simulink model "BMS_4S1P"  (R2026a)
settings: Solver=VariableStepAuto  StopTime=600
libraries: fl_lib x20, nesl_utility x15, simulink x3, BMS_4S1P_ExternalBalancing_lib_lib x1, BatteryBalancing x1, BatteryEstimators x1
settings Model: Creator=jack2  LastModifiedBy=jack2

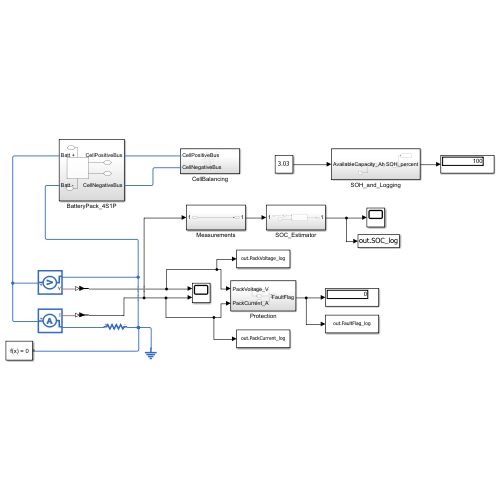
[thumbnail: Simulink's stored preview of the top-level diagram]
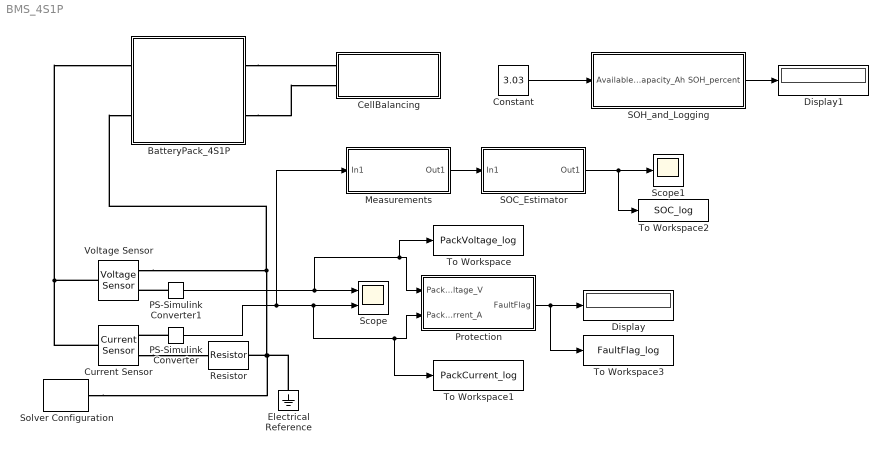
== system BMS_4S1P ==
  BatteryPack_4S1P : Subsystem
  CellBalancing : Subsystem
  Constant : Constant  Value=3.03
  Current Sensor : fl_lib/Electrical/Electrical Sensors/Current Sensor
  Display : Display
  Display1 : Display
  Electrical Reference : fl_lib/Electrical/Electrical Elements/Electrical Reference
  Measurements : Subsystem
  PS-Simulink Converter : nesl_utility/PS-Simulink Converter  PhysicalDomain=network_engine_domain  SubClassName=ps_output  LeftPortType=input  RightPortType=output  PseudoPeriodic=off  Frequencies=[]  VectorFormat=inherit  Unit=A  AffineConversion=off
  PS-Simulink Converter1 : nesl_utility/PS-Simulink Converter  PhysicalDomain=network_engine_domain  SubClassName=ps_output  LeftPortType=input  RightPortType=output  PseudoPeriodic=off  Frequencies=[]  VectorFormat=inherit  Unit=V  AffineConversion=off
  Protection : Subsystem
  Resistor : fl_lib/Electrical/Electrical Elements/Resistor  R=20 Ohm  i_specify=off  i_priority=None  i=0 A  i_nominal_specify=off  i_nominal_value=1  i_nominal_unit=A  v_specify=off  v_priority=None  v=0 V  v_nominal_specify=off  v_nominal_value=1  v_nominal_unit=V
  SOC_Estimator : Subsystem
  SOH_and_Logging : Subsystem
  Scope : Scope  NumInputPorts=2
      settings: ActiveDisplayYMinimum=2.7734819938047579  ActiveDisplayYMaximum=17.948779649470726
  Scope1 : Scope
      settings: ActiveDisplayYMinimum=0.77520540586084219  ActiveDisplayYMaximum=0.832743677575157
  Solver Configuration : nesl_utility/Solver Configuration  PhysicalDomain=network_engine_domain  SubClassName=solver  LeftPortType=input  RightPortType=generic  Tones=[]  Harmonics=[]  SimulateNoise=off  Profile=off  UseLocalSampling=off  EnableSwitchedLinearOptims=on  FrequencyDomain=off  UseCCode=off  RelTol=0.001  AbsTol=0.001  MinStep=1e-09  ToWorkspace=off  RevertToSquareIcSolve=off  NumHomotopyIterations=100  PhasorMode=off  PhasorModeNumHarmonics=1  ConsistencySolver=NEWTON_XTOL_AFTER_FTOL  CanonicalOrdering=CANONICAL  OptimizeIntermediates=OPTIMIZED  IndexReductionMethod=DerivativeReplacement  DoDC=off  ResidualTolerance=1e-09  ConsistencyTolSource=GLOBAL  ConsistencyAbsTol=0.001  ConsistencyRelTol=0.001  ConsistencyTolFactor=0.001  UseLocalSolver=off  LocalSolverChoice=NE_BACKWARD_EULER_ADVANCER  ResolveIndetEquations=on  FunctionEvalNumThread=1  LocalSolverSampleTime=0.001  DoFixedCost=off  MaxNonlinIter=3  MaxModeIter=2  ComputeImpulses=off  ImpulseIterations=2  LinearAlgebra=auto  LinearAlgebraNumThread=0  EquationFormulation=NE_TIME_EF  DelaysMemoryBudget=1024  AutomaticFiltering=on  FilteringTimeConstant=0.001  PartitionStorageMethod=AS_NEEDED  PartitionMemoryBudget=1024  PartitionMethod=ROBUST  MultibodyUseLocalSolver=off  MultibodyLocalSolverChoice=ODE1  MultibodyLocalSolverSampleTime=0.001
  To Workspace : ToWorkspace  VariableName=PackVoltage_log  SaveFormat=Timeseries  SampleTime=-1
  To Workspace1 : ToWorkspace  VariableName=PackCurrent_log  SaveFormat=Timeseries  SampleTime=-1
  To Workspace2 : ToWorkspace  VariableName=SOC_log  SaveFormat=Timeseries  SampleTime=-1
  To Workspace3 : ToWorkspace  VariableName=FaultFlag_log  SaveFormat=Timeseries  SampleTime=-1
  Voltage Sensor : fl_lib/Electrical/Electrical Sensors/Voltage Sensor
  wires:
  Measurements/1(Out1) -> SOC_Estimator/1(In1)
  PS-Simulink Converter/1 -> Measurements/1(In1), Scope/2, To Workspace1/1, Protection/2(PackCurrent_A)
  PS-Simulink Converter1/1 -> To Workspace/1, Protection/1(PackVoltage_V), Scope/1
  SOC_Estimator/1(Out1) -> To Workspace2/1, Scope1/1
  Protection/1(FaultFlag) -> To Workspace3/1, Display/1
  Constant/1 -> SOH_and_Logging/1(AvailableCapacity_Ah)
  SOH_and_Logging/1(SOH_percent) -> Display1/1
  connections:
  Current Sensor/LConn1 -- BatteryPack_4S1P/LConn1 -- Voltage Sensor/LConn1
  Current Sensor/RConn2 -- Resistor/LConn1
  Solver Configuration/RConn1 -- Electrical Reference/LConn1 -- BatteryPack_4S1P/LConn2 -- Voltage Sensor/RConn2 -- Resistor/RConn1
  PS-Simulink Converter1/LConn1 -- Voltage Sensor/RConn1
  PS-Simulink Converter/LConn1 -- Current Sensor/RConn1
  BatteryPack_4S1P/RConn1 -- CellBalancing/LConn1
  BatteryPack_4S1P/RConn2 -- CellBalancing/LConn2

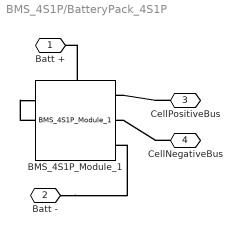
== system BMS_4S1P/BatteryPack_4S1P ==
  BMS_4S1P_Module_1 : BMS_4S1P_ExternalBalancing_lib_lib/BMS_4S1P_Module_1  SOC_vecCell=[0, .01, .02, .03, .04, .05, .06, .07, .08, .09, .1, .11, .12, .13, .14, .15, .16, .17, .18, .19, .2, .21, .22, .23, .24, .25, .26, .27, .28, .29, .3, .31, .32, .33, .34, .35, .36, .37, .38, .39, .4, .41, .42, .43, .44, .45, .46, .47, .48, .49, .5, .51, .52, .53, .54, .55, .56, .57, .58, .59, .6, .61, .62, .63, .64, .65, .66, .67, .68, .69, .7, .71, .72, .73, .74, .75, .76, .77, .78, .79, .8, .81, .82, .83, .84, .85, .86, .87, .88, .89, .9, .91, .92, .93, .94, .95, .96, .97, .98, .99, 1]  V0_vecCell=[2.90003, 2.94341, 2.98679, 3.04987, 3.09433, 3.12791, 3.16031, 3.20369, 3.23862, 3.26689, 3.29115, 3.31383, 3.33202, 3.35112, 3.36833, 3.38413, 3.39973, 3.41137, 3.42149, 3.43136, 3.44073, 3.45027, 3.46068, 3.47113, 3.47814, 3.48494, 3.49199, 3.49905, 3.50562, 3.51187, 3.51861, 3.52535, 3.53209, 3.53818, 3.54353, 3.54849, 3.55353, 3.55855, 3.56357, 3.56831, 3.57308, 3.57787, 3.58264, 3.58755, 3.5925, 3.5985, 3.60496, 3.61149, 3.61805, 3.6246, 3.63116, 3.63855, 3.64609, 3.65336, 3.66064, 3.66791, 3.67613, 3.68522, 3.69443, 3.70367, 3.713, 3.72241, 3.73154, 3.74037, 3.7492, 3.75786, 3.76617, 3.77556, 3.78485, 3.79413, 3.8034, 3.81149, 3.81977, 3.82804, 3.83631, 3.84472, 3.85317, 3.86155, 3.86993, 3.87831, 3.88686, 3.89534, 3.90461, 3.91454, 3.92565, 3.93721, 3.94924, 3.96155, 3.97383, 3.98598, 3.99856, 4.01117, 4.02361, 4.03609, 4.04694, 4.05695, 4.06641, 4.07551, 4.08514, 4.09447, 4.10453] V  V_rangeCell=[2.25, Inf] V  R0_vecCell=[.1741, .15823, .14313, .13285, .12044, .10641, .09605, .09162, .08758, .08349, .08021, .07738, .07487, .07338, .07189, .07117, .0704, .06898, .06755, .06631, .06509, .06388, .06326, .06281, .06182, .06095, .06025, .05955, .05877, .05807, .05761, .05714, .05668, .05611, .05546, .0549, .05439, .05388, .05337, .0528, .05223, .05165, .05106, .05046, .04986, .04945, .04913, .04883, .04854, .04826, .04797, .04782, .04765, .0473, .04695, .04661, .04638, .0463, .04625, .04621, .04624, .04628, .04628, .04623, .04617, .04599, .04573, .0457, .04568, .04565, .04563, .04535, .0451, .04486, .04461, .04446, .04435, .04423, .04411, .044, .04372, .04339, .04323, .0432, .04344, .04374, .0441, .04452, .04494, .0454, .04594, .0463, .04649, .04668, .04629, .04541, .04438, .04326, .04154, .03869, .03326] Ohm  AHCell=3.03 A*hr  extrapolation_optionCell=simscape.enum.extrapolation.nearest  iCell_specify=off  iCell_priority=None  iCell=repmat(0, 4, 1) A  iCell_nominal_specify=off  iCell_nominal_value=1  iCell_nominal_unit=A  vCell_specify=off  vCell_priority=None  vCell=repmat(0, 4, 1) V  vCell_nominal_specify=off  vCell_nominal_value=1  vCell_nominal_unit=V  socCell_specify=on  socCell_priority=High  socCell=[0.90;0.80;0.50;0.80]  socCell_nominal_specify=off  socCell_nominal_value=1  socCell_nominal_unit=1  numCyclesCell_specify=off  numCyclesCell_priority=High  numCyclesCell=repmat(0, 4, 1)  numCyclesCell_nominal_specify=off  numCyclesCell_nominal_value=1  numCyclesCell_nominal_unit=1  vParallelAssembly_specify=off  vParallelAssembly_priority=None  vParallelAssembly=repmat(0, 4, 1) V  vParallelAssembly_nominal_specify=off  vParallelAssembly_nominal_value=1  vParallelAssembly_nominal_unit=V  socParallelAssembly_specify=off  socParallelAssembly_priority=None  socParallelAssembly=repmat(1, 4, 1)  socParallelAssembly_nominal_specify=off  socParallelAssembly_nominal_value=1  socParallelAssembly_nominal_unit=1
  Batt + : PMIOPort  Side=Left
  Batt - : PMIOPort  Port=2  Side=Left
  CellPositiveBus : PMIOPort  Port=3  Side=Right
  CellNegativeBus : PMIOPort  Port=4  Side=Right
  connections:
  BMS_4S1P_Module_1/LConn1 -- Batt +/RConn1
  Batt -/RConn1 -- BMS_4S1P_Module_1/RConn3
  CellPositiveBus/RConn1 -- BMS_4S1P_Module_1/RConn1
  CellNegativeBus/RConn1 -- BMS_4S1P_Module_1/RConn2

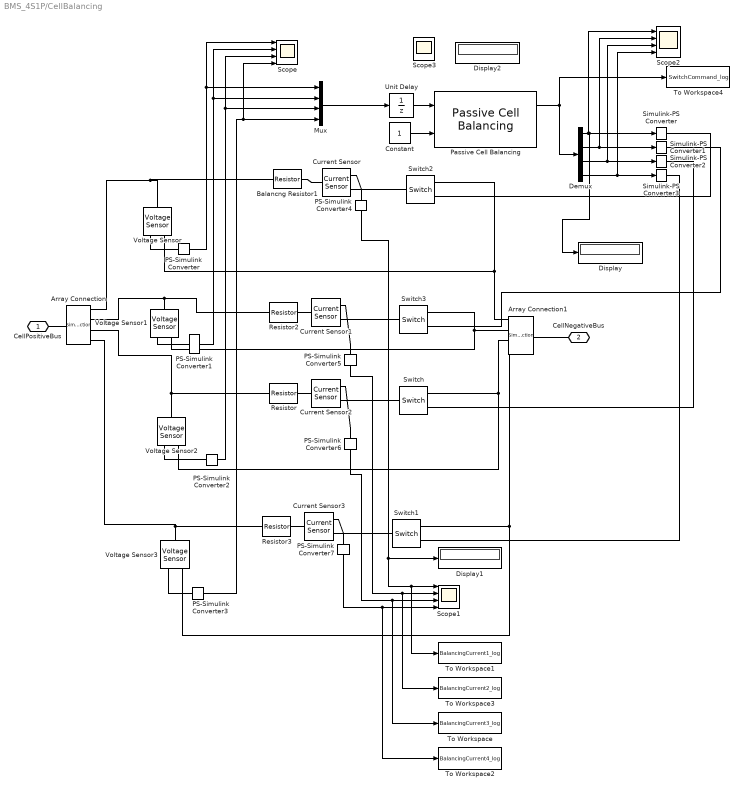
== system BMS_4S1P/CellBalancing ==
  Array Connection : SimscapeArrayConnection  NumScalarElements=4
  Array Connection1 : SimscapeArrayConnection  NumScalarElements=4
  Balancng Resistor1 : fl_lib/Electrical/Electrical Elements/Resistor  R=82 Ohm  i_specify=off  i_priority=None  i=0 A  i_nominal_specify=off  i_nominal_value=1  i_nominal_unit=A  v_specify=off  v_priority=None  v=0 V  v_nominal_specify=off  v_nominal_value=1  v_nominal_unit=V
  Constant : Constant
  Current Sensor{,1..3} (4 alike) : fl_lib/Electrical/Electrical Sensors/Current Sensor
  Demux : Demux
  Display : Display
  Display1 : Display
  Display2 : Display
  Mux : Mux
  PS-Simulink Converter{,1..3} (4 alike) : nesl_utility/PS-Simulink Converter  PhysicalDomain=network_engine_domain  SubClassName=ps_output  LeftPortType=input  RightPortType=output  PseudoPeriodic=off  Frequencies=[]  VectorFormat=inherit  Unit=V  AffineConversion=off
  PS-Simulink Converter{4..7} (4 alike) : nesl_utility/PS-Simulink Converter  PhysicalDomain=network_engine_domain  SubClassName=ps_output  LeftPortType=input  RightPortType=output  PseudoPeriodic=off  Frequencies=[]  VectorFormat=inherit  Unit=A  AffineConversion=off
  Passive Cell Balancing : BatteryBalancing/Passive Cell Balancing  Threshold=0.02  HysteresisBand=0.005  Td_on=1  Td_off=1  Ts=1  dataType=double
      settings: LibrarySourceBlock=batt_sl_lib/Cell Balancing/Passive Cell Balancing
  Resistor : fl_lib/Electrical/Electrical Elements/Resistor  R=82 Ohm  i_specify=off  i_priority=None  i=0 A  i_nominal_specify=off  i_nominal_value=1  i_nominal_unit=A  v_specify=off  v_priority=None  v=0 V  v_nominal_specify=off  v_nominal_value=1  v_nominal_unit=V
  Resistor2 : fl_lib/Electrical/Electrical Elements/Resistor  R=82 Ohm  i_specify=off  i_priority=None  i=0 A  i_nominal_specify=off  i_nominal_value=1  i_nominal_unit=A  v_specify=off  v_priority=None  v=0 V  v_nominal_specify=off  v_nominal_value=1  v_nominal_unit=V
  Resistor3 : fl_lib/Electrical/Electrical Elements/Resistor  R=82 Ohm  i_specify=off  i_priority=None  i=0 A  i_nominal_specify=off  i_nominal_value=1  i_nominal_unit=A  v_specify=off  v_priority=None  v=0 V  v_nominal_specify=off  v_nominal_value=1  v_nominal_unit=V
  Scope : Scope  NumInputPorts=4
      settings: ActiveDisplayYMinimum=3.9018352664454508  ActiveDisplayYMaximum=3.9703474561372  DataLoggingVariableName=ScopeData2
  Scope1 : Scope  NumInputPorts=4
      settings: ActiveDisplayYMinimum=-0.0026801401894574819  ActiveDisplayYMaximum=0.12126798116461307  DataLoggingVariableName=ScopeData3
  Scope2 : Scope  NumInputPorts=4
      settings: ActiveDisplayYMinimum=-0.17607488610478361  ActiveDisplayYMaximum=1.2020501138952164  DataLoggingVariableName=ScopeData4
  Scope3 : Scope
      settings: ActiveDisplayYMinimum=-1  ActiveDisplayYMaximum=1  DataLoggingVariableName=ScopeData5
  Simulink-PS Converter{,1..3} (4 alike) : nesl_utility/Simulink-PS Converter  PhysicalDomain=network_engine_domain  SubClassName=ps_input  LeftPortType=input  RightPortType=output  PseudoPeriodic=off  Frequencies=[]  NoiseDistribution=none  NoiseParameters=[]  Unit=1  AffineConversion=off  FilteringAndDerivatives=provide  SimscapeFilterOrder=1  InputFilterTimeConstant=0.001  UdotUserProvided=0
  Switch{,1..3} (4 alike) : fl_lib/Electrical/Electrical Elements/Switch  R_closed=0.01 Ohm  G_open=1e-8 1/Ohm  Threshold=0.5  i_specify=off  i_priority=None  i=0 A  i_nominal_specify=off  i_nominal_value=1  i_nominal_unit=A  v_specify=off  v_priority=None  v=0 V  v_nominal_specify=off  v_nominal_value=1  v_nominal_unit=V
  To Workspace : ToWorkspace  VariableName=BalancingCurrent3_log  SaveFormat=Timeseries  SampleTime=-1
  To Workspace1 : ToWorkspace  VariableName=BalancingCurrent1_log  SaveFormat=Timeseries  SampleTime=-1
  To Workspace2 : ToWorkspace  VariableName=BalancingCurrent4_log  SaveFormat=Timeseries  SampleTime=-1
  To Workspace3 : ToWorkspace  VariableName=BalancingCurrent2_log  SaveFormat=Timeseries  SampleTime=-1
  To Workspace4 : ToWorkspace  VariableName=SwitchCommand_log  SaveFormat=Timeseries  SampleTime=-1
  Unit Delay : UnitDelay  InitialCondition=4.08  SampleTime=-1
  Voltage Sensor{,1..3} (4 alike) : fl_lib/Electrical/Electrical Sensors/Voltage Sensor
  CellPositiveBus : PMIOPort  Side=Left
  CellNegativeBus : PMIOPort  Port=2  Side=Left
  wires:
  PS-Simulink Converter/1 -> Scope/1, Mux/1
  PS-Simulink Converter1/1 -> Mux/2, Scope/2
  PS-Simulink Converter2/1 -> Mux/3, Scope/3
  PS-Simulink Converter3/1 -> Mux/4, Scope/4
  Unit Delay/1 -> Passive Cell Balancing/1
  Constant/1 -> Passive Cell Balancing/2
  Mux/1 -> Unit Delay/1
  Passive Cell Balancing/1 -> Demux/1, To Workspace4/1
  Demux/1 -> Scope2/1, Simulink-PS Converter/1, Display/1
  Demux/2 -> Scope2/2, Simulink-PS Converter1/1
  Demux/3 -> Scope2/3, Simulink-PS Converter2/1
  Demux/4 -> Scope2/4, Simulink-PS Converter3/1
  PS-Simulink Converter4/1 -> To Workspace1/1, Scope1/1, Display1/1
  PS-Simulink Converter5/1 -> To Workspace3/1, Scope1/2
  PS-Simulink Converter6/1 -> To Workspace/1, Scope1/3
  PS-Simulink Converter7/1 -> To Workspace2/1, Scope1/4
  connections:
  Array Connection/RConn1 -- CellPositiveBus/RConn1
  CellNegativeBus/RConn1 -- Array Connection1/RConn1
  Voltage Sensor1/LConn1 -- Array Connection/LConn2 -- Resistor2/LConn1
  Voltage Sensor2/LConn1 -- Array Connection/LConn3 -- Resistor/LConn1
  Voltage Sensor3/LConn1 -- Resistor3/LConn1 -- Array Connection/LConn4
  PS-Simulink Converter1/LConn1 -- Voltage Sensor1/RConn1
  PS-Simulink Converter/LConn1 -- Voltage Sensor/RConn1
  PS-Simulink Converter2/LConn1 -- Voltage Sensor2/RConn1
  PS-Simulink Converter3/LConn1 -- Voltage Sensor3/RConn1
  Switch/RConn2 -- Voltage Sensor2/RConn2 -- Array Connection1/LConn3
  Switch1/RConn2 -- Voltage Sensor3/RConn2 -- Array Connection1/LConn4
  Switch3/RConn2 -- Voltage Sensor1/RConn2 -- Array Connection1/LConn2
  Array Connection/LConn1 -- Voltage Sensor/LConn1 -- Balancng Resistor1/LConn1
  Switch2/RConn2 -- Array Connection1/LConn1 -- Voltage Sensor/RConn2
  Simulink-PS Converter1/RConn1 -- Switch3/RConn1
  Simulink-PS Converter2/RConn1 -- Switch/RConn1
  Simulink-PS Converter3/RConn1 -- Switch1/RConn1
  PS-Simulink Converter4/LConn1 -- Current Sensor/RConn1
  Current Sensor/LConn1 -- Balancng Resistor1/RConn1
  Current Sensor/RConn2 -- Switch2/LConn1
  PS-Simulink Converter5/LConn1 -- Current Sensor1/RConn1
  Current Sensor1/RConn2 -- Switch3/LConn1
  Resistor2/RConn1 -- Current Sensor1/LConn1
  PS-Simulink Converter6/LConn1 -- Current Sensor2/RConn1
  Current Sensor2/RConn2 -- Switch/LConn1
  Resistor/RConn1 -- Current Sensor2/LConn1
  PS-Simulink Converter7/LConn1 -- Current Sensor3/RConn1
  Current Sensor3/RConn2 -- Switch1/LConn1
  Resistor3/RConn1 -- Current Sensor3/LConn1
  Simulink-PS Converter/RConn1 -- Switch2/RConn1

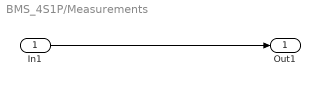
== system BMS_4S1P/Measurements ==
  In1 : Inport
  Out1 : Outport
  wires:
  In1/1 -> Out1/1

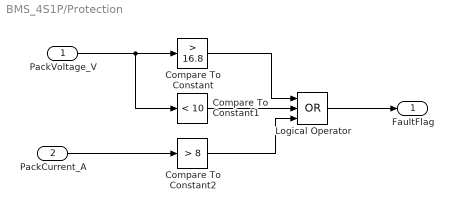
== system BMS_4S1P/Protection ==
  PackVoltage_V : Inport
  PackCurrent_A : Inport  Port=2
  Compare To Constant : simulink/Logic and Bit Operations/Compare To Constant  relop=>  const=16.8  OutDataTypeStr=boolean
  Compare To Constant1 : simulink/Logic and Bit Operations/Compare To Constant  relop=<  const=10  OutDataTypeStr=boolean
  Compare To Constant2 : simulink/Logic and Bit Operations/Compare To Constant  relop=>  const=8  OutDataTypeStr=boolean
  Logical Operator : Logic  Operator=OR  Inputs=3  AllPortsSameDT=off  OutDataTypeStr=boolean
  FaultFlag : Outport
  wires:
  PackVoltage_V/1 -> Compare To Constant1/1, Compare To Constant/1
  PackCurrent_A/1 -> Compare To Constant2/1
  Compare To Constant/1 -> Logical Operator/1
  Compare To Constant1/1 -> Logical Operator/2
  Compare To Constant2/1 -> Logical Operator/3
  Logical Operator/1 -> FaultFlag/1

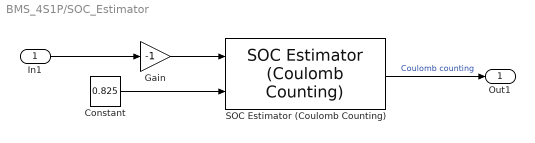
== system BMS_4S1P/SOC_Estimator ==
  In1 : Inport
  Constant : Constant  Value=0.825
  Gain : Gain  Gain=-1
  SOC Estimator (Coulomb Counting) : BatteryEstimators/SOC Estimator (Coulomb Counting)  CurrentInputPartition=off  AH=3.03  Ts=1  DataType=Inherit: auto
      settings: LibrarySourceBlock=|
      | batt_sl_lib/Estimators/SOC Estimator
      | (Coulomb Counting)
  Out1 : Outport
  wires:
  In1/1 -> Gain/1
  Gain/1 -> SOC Estimator (Coulomb Counting)/1
  Constant/1 -> SOC Estimator (Coulomb Counting)/2
  SOC Estimator (Coulomb Counting)/1 -> Out1/1  "Coulomb counting"

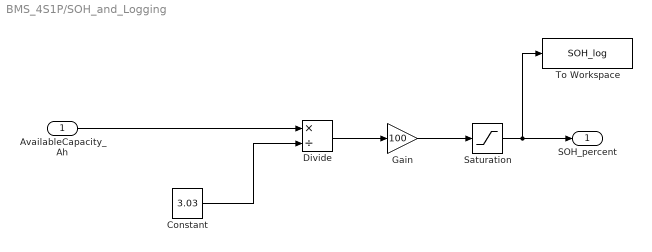
== system BMS_4S1P/SOH_and_Logging ==
  AvailableCapacity_Ah : Inport
  Constant : Constant  Value=3.03
  Divide : Product  Inputs=*/
  Gain : Gain  Gain=100
  Saturation : Saturate  UpperLimit=100  LowerLimit=0
  To Workspace : ToWorkspace  VariableName=SOH_log  SaveFormat=Timeseries  SampleTime=-1
  SOH_percent : Outport
  wires:
  AvailableCapacity_Ah/1 -> Divide/1
  Constant/1 -> Divide/2
  Divide/1 -> Gain/1
  Gain/1 -> Saturation/1
  Saturation/1 -> SOH_percent/1, To Workspace/1
